simulink model "scheme_L2"  (R2025b)
settings: Solver=VariableStepAuto  StartTime=0.0  StopTime=10  RelTol=1e-3
settings Model: Creator=yzhar  LastModifiedBy=semzi

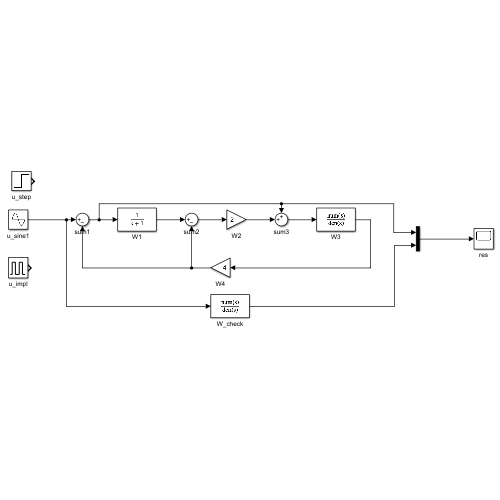
[thumbnail: Simulink's stored preview of the top-level diagram]
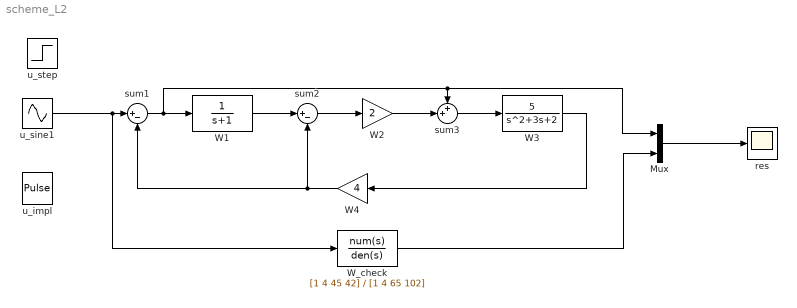
== system scheme_L2 ==
  Mux : Mux  Inputs=2
  W1 : TransferFcn  Denominator=[1 1]
  W2 : Gain  Gain=2
  W3 : TransferFcn  Numerator=[5]  Denominator=[1 3 2]
  W4 : Gain  Gain=4
  W_check : TransferFcn  Numerator=[1 4 45 42]  Denominator=[1 4 65 102]
  res : Scope
      settings: ActiveDisplayYMinimum=-0.72877080280283146  ActiveDisplayYMaximum=0.7193403590156765
  sum1 : Sum  Inputs=|+-
  sum2 : Sum  Inputs=|+-
  sum3 : Sum  Inputs=++|
  u_impl : DiscretePulseGenerator  PulseType=Time based  Amplitude=20  Period=20  PulseWidth=0.05  PhaseDelay=1
  u_sine1 : Sin  Frequency=2  SampleTime=0
  u_step : Step  SampleTime=0
  wires:
  u_sine1/1 -> W_check/1, sum1/1
  sum1/1 -> W1/1, Mux/1, sum3/1
  sum2/1 -> W2/1
  W2/1 -> sum3/2
  sum3/1 -> W3/1
  W3/1 -> W4/1
  W4/1 -> sum2/2, sum1/2
  Mux/1 -> res/1
  W1/1 -> sum2/1
  W_check/1 -> Mux/2
